simulink model "ProgettoIT"  (R2026b)
settings: Solver=VariableStepAuto  StopTime=3657
values from neighbouring files (symbols this model uses):
  m = sum(v .* dt) / Tstop    [excel.m]
  n = zeros(7,1)    [excel.m]
settings Model: Creator=francescocavazzoli  LastModifiedBy=Lorenzo

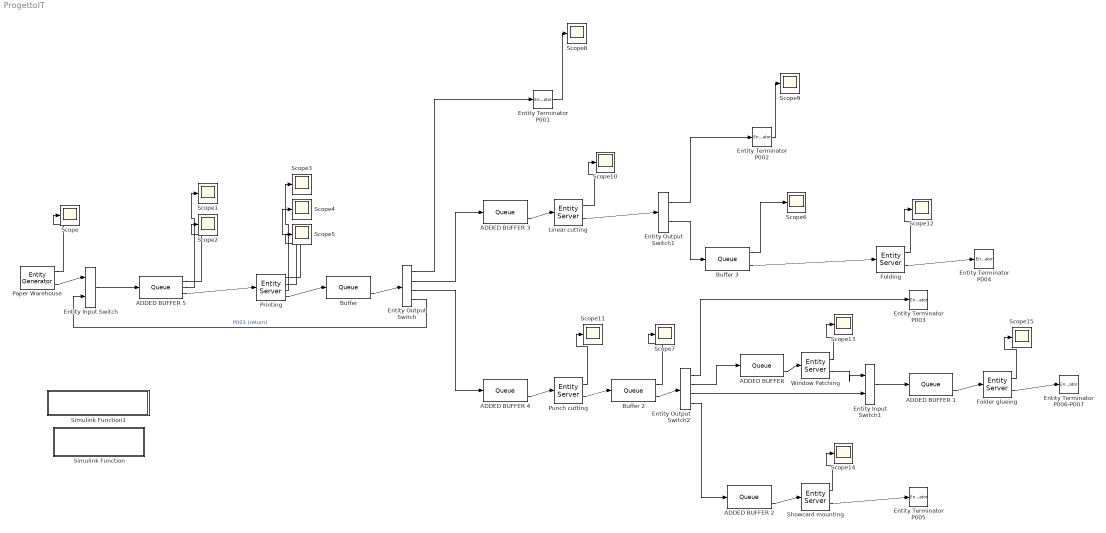
== system ProgettoIT ==
  ADDED BUFFER : Queue  InputPortMessageModes=m  OutputPortMessageModes=n,m  Capacity=inf  NumberEntitiesInBlock=on
      settings: OutputPortMap=o1,o5
  ADDED BUFFER {1..4} (4 alike) : Queue  InputPortMessageModes=m  OutputPortMessageModes=n,m  Capacity=inf  NumberEntitiesInBlock=on
      settings: OutputPortMap=o1,o5
  ADDED BUFFER 5 : Queue  InputPortMessageModes=m  OutputPortMessageModes=n,n,m  Capacity=inf  NumberEntitiesDeparted=on  NumberEntitiesInBlock=on
      settings: OutputPortMap=o0,o1,o5
  Buffer : Queue  InputPortMessageModes=m  OutputPortMessageModes=n,m  Capacity=inf  SortingDirection=Descending  NumberEntitiesInBlock=on
      settings: OutputPortMap=o1,o5
  Buffer 2 : Queue  InputPortMessageModes=m  OutputPortMessageModes=n,m  Capacity=inf  NumberEntitiesInBlock=on
      settings: OutputPortMap=o1,o5
  Buffer 3 : Queue  InputPortMessageModes=m  OutputPortMessageModes=n,m  Capacity=inf  NumberEntitiesInBlock=on
      settings: OutputPortMap=o1,o5
  Entity Input Switch : EntityInputSwitch  InputPortMessageModes=m,m  OutputPortMessageModes=m
  Entity Input Switch1 : EntityInputSwitch  InputPortMessageModes=m,m  OutputPortMessageModes=m
  Entity Output Switch : EntityOutputSwitch  InputPortMessageModes=m  OutputPortMessageModes=m,m,m,m  NumberOutputPorts=4  SwitchingCriterion=From attribute  SwitchAttributeName=OutPrint
      settings: OutputPortMap=o0,o1,o2,o3
  Entity Output Switch1 : EntityOutputSwitch  InputPortMessageModes=m  OutputPortMessageModes=m,m  SwitchingCriterion=From attribute  SwitchAttributeName=OutLin
  Entity Output Switch2 : EntityOutputSwitch  InputPortMessageModes=m  OutputPortMessageModes=m,m,m,m  NumberOutputPorts=4  SwitchingCriterion=From attribute  SwitchAttributeName=OutPunch
      settings: OutputPortMap=o0,o1,o2,o3
  Entity Terminator P001 : EntityTerminator  InputPortMessageModes=m  EntryAction=|  NumberEntitiesArrived=on
      | entity.FlowTime = ReadTime() - entity.Arrival;      % tempo di attraversamento [h]
      | Late = max(0, ReadTime() - entity.DueDate);          % ritardo rispetto al tempo max [h]
      | ToWorkspace(entity.Type, entity.FlowTime, Late);
      settings: OutputPortMap=o0
  Entity Terminator P002 : EntityTerminator  InputPortMessageModes=m  EntryAction=|  NumberEntitiesArrived=on
      | entity.FlowTime = ReadTime() - entity.Arrival;      % tempo di attraversamento [h]
      | Late = max(0, ReadTime() - entity.DueDate);          % ritardo rispetto al tempo max [h]
      | ToWorkspace(entity.Type, entity.FlowTime, Late);
      settings: OutputPortMap=o0
  "Entity Terminator P003 " : EntityTerminator  InputPortMessageModes=m  EntryAction=|
      | entity.FlowTime = ReadTime() - entity.Arrival;      % tempo di attraversamento [h]
      | Late = max(0, ReadTime() - entity.DueDate);          % ritardo rispetto al tempo max [h]
      | ToWorkspace(entity.Type, entity.FlowTime, Late);
  Entity Terminator P004 : EntityTerminator  InputPortMessageModes=m  EntryAction=|
      | entity.FlowTime = ReadTime() - entity.Arrival;      % tempo di attraversamento [h]
      | Late = max(0, ReadTime() - entity.DueDate);          % ritardo rispetto al tempo max [h]
      | ToWorkspace(entity.Type, entity.FlowTime, Late);
  "Entity Terminator P005 " : EntityTerminator  InputPortMessageModes=m  EntryAction=|
      | entity.FlowTime = ReadTime() - entity.Arrival;      % tempo di attraversamento [h]
      | Late = max(0, ReadTime() - entity.DueDate);          % ritardo rispetto al tempo max [h]
      | ToWorkspace(entity.Type, entity.FlowTime, Late);
  "Entity Terminator P006-P007 " : EntityTerminator  InputPortMessageModes=m  EntryAction=|
      | entity.FlowTime = ReadTime() - entity.Arrival;      % tempo di attraversamento [h]
      | Late = max(0, ReadTime() - entity.DueDate);          % ritardo rispetto al tempo max [h]
      | ToWorkspace(entity.Type, entity.FlowTime, Late);
  Folder glueing : EntityServer  InputPortMessageModes=m  OutputPortMessageModes=n,m  Capacity=2  ServiceTimeSource=MATLAB action  ServiceTimeAction=dt = (4 + entity.Pieces/54000)/0.5293;  Utilization=on
      settings: OutputPortMap=o5,o9
  Folding : EntityServer  InputPortMessageModes=m  OutputPortMessageModes=n,m  Capacity=3  ServiceTimeSource=MATLAB action  ServiceTimeAction=dt = (4 + entity.Pieces/5000)/0.5293;  Utilization=on
      settings: OutputPortMap=o5,o9
  Linear cutting : EntityServer  InputPortMessageModes=m  OutputPortMessageModes=n,m  Capacity=1  ServiceTimeSource=MATLAB action  ServiceTimeAction=dt = (0.5 + entity.Pieces/180000)/0.5293;  Utilization=on
      settings: OutputPortMap=o5,o9
  Paper Warehouse : EntityGenerator  OutputPortMessageModes=n,m  TimeSource=MATLAB action  IntergenerationTimeAction=|  GenerateAction=|  AttributeName=Pieces|Sheets|Type|Arrival|Pass|DueDate|OutPrint|OutLin|OutPunch|FlowTime  AttributeInitialValue=0|0|0|0|0|0|0|0|0|0  NumberEntitiesDeparted=on  EntityType=Structured  EntityTypeName=Entity
      IntergenerationTimeAction=|
      | coder.extrinsic('exprnd');
      | dt = 0.0; % Pre-allocazione per il compilatore
      | dt = exprnd(3657/600);
      GenerateAction=|
      | coder.extrinsic('randsample');
      | P = [0.15 0.03 0.42 0.04 0.05 0.23 0.08];        % % ordini P001..P007
      | S = [53333 53333 26667 50000 40000 24348 120000]; % fogli per ordine
      | T = [90 90 90 435 165 135 360];                   % tempo max di attraversamento [h]
      | type_val = 0; % Pre-allocazione per il compilatore
      | type_val = randsample(1:7, 1, true, P);
      | entity.Type = type_val;
      | entity.Sheets  = S(entity.Type);
      | entity.Pieces  = 18*entity.Sheets;
      | entity.Pass    = 0;
      | entity.Arrival = ReadTime();
      | entity.DueDate = entity.Arrival + T(entity.Type);
      | LP = [0 1 0 2 0 0 0];  entity.OutLin   = LP(entity.Type);  % dopo il taglio lineare: 1 = fine, 2 = piega
      | PU = [0 0 1 0 4 3 2];  entity.OutPunch = PU(entity.Type);  % dopo la fustella: 1 = fine, 2 = Finestratura, 3 = piega-incolla, 4 = owo
      settings: OutputPortMap=o0,o3
  Printing : EntityServer  InputPortMessageModes=m  OutputPortMessageModes=n,n,n,m  Capacity=3  ServiceTimeSource=MATLAB action  ServiceTimeValue=1/8000  ServiceTimeAction=dt = (5*20/60 + entity.Sheets/8000)/0.5293;  ServiceCompleteAction=|  NumberEntitiesDeparted=on  NumberEntitiesInBlock=on  Utilization=on
      | entity.Pass = entity.Pass + 1;
      | if entity.Type == 1 && entity.Pass == 1
      |     entity.OutPrint = 4;      % P001: ritorno in stampa
      | elseif entity.Type == 1
      |     entity.OutPrint = 1;      % P001 finito
      | elseif entity.Type == 2 || entity.Type == 4
      |     entity.OutPrint = 2;      % taglio lineare
      | else
      |     entity.OutPrint = 3;      % fustella
      | end
      settings: OutputPortMap=o0,o1,o5,o9
  "Punch cutting " : EntityServer  InputPortMessageModes=m  OutputPortMessageModes=n,m  Capacity=3  ServiceTimeSource=MATLAB action  ServiceTimeAction=dt = (2 + entity.Sheets/4000)/0.5293;  Utilization=on
      settings: OutputPortMap=o5,o9
  Scope{,1..15} (16 alike) : Scope
      Scope settings: ActiveDisplayYMinimum=-0.99999999999999956  ActiveDisplayYMaximum=19
      Scope10 settings: ActiveDisplayYMinimum=-0.024471490848986532  ActiveDisplayYMaximum=0.44643519443886448  DataLoggingVariableName=ScopeData10
      Scope11 settings: DataLoggingVariableName=ScopeData11
      Scope12 settings: ActiveDisplayYMinimum=0.25497380327143887  ActiveDisplayYMaximum=0.75796557224527028  DataLoggingVariableName=ScopeData12
      Scope13 settings: ActiveDisplayYMinimum=0.40962558539871696  ActiveDisplayYMaximum=0.68711566304961347  DataLoggingVariableName=ScopeData13
      Scope14 settings: ActiveDisplayYMinimum=0.075905038165493571  ActiveDisplayYMaximum=0.25791292970081553  DataLoggingVariableName=ScopeData14
      Scope15 settings: DataLoggingVariableName=ScopeData15
      Scope2 settings: DataLoggingVariableName=ScopeData2
      Scope3 settings: ActiveDisplayYMinimum=0.2405445003600471  ActiveDisplayYMaximum=1.0583804541198938  DataLoggingVariableName=ScopeData3
      Scope4 settings: DataLoggingVariableName=ScopeData4
      Scope5 settings: DataLoggingVariableName=ScopeData5
      Scope6 settings: DataLoggingVariableName=ScopeData6
      Scope7 settings: DataLoggingVariableName=ScopeData7
      Scope8 settings: DataLoggingVariableName=ScopeData8
      Scope9 settings: DataLoggingVariableName=ScopeData9
  Showcard mounting : EntityServer  InputPortMessageModes=m  OutputPortMessageModes=n,m  Capacity=1  ServiceTimeSource=MATLAB action  ServiceTimeAction=dt = (4 + entity.Pieces/54000)/0.5293;  Utilization=on
      settings: OutputPortMap=o5,o9
  Simulink Function : Subsystem  TreatAsAtomicUnit=on
  Simulink Function1 : Subsystem  TreatAsAtomicUnit=on
  Window Patching : EntityServer  InputPortMessageModes=m  OutputPortMessageModes=n,m  Capacity=2  ServiceTimeSource=MATLAB action  ServiceTimeAction=dt = (4 + entity.Pieces/54000)/0.5293;  Utilization=on
      settings: OutputPortMap=o5,o9
  wires:
  Printing/4 -> Buffer/1
  Buffer/2 -> Entity Output Switch/1
  Entity Output Switch/1 -> Entity Terminator P001/1
  Entity Output Switch/2 -> ADDED BUFFER 3/1
  Entity Output Switch/3 -> ADDED BUFFER 4/1
  Entity Output Switch/4 -> Entity Input Switch/2  "P001 (return)"
  Buffer 3/2 -> Folding/1
  Linear cutting/2 -> Entity Output Switch1/1
  Entity Output Switch1/2 -> Buffer 3/1
  Entity Output Switch1/1 -> Entity Terminator P002/1
  Entity Output Switch2/1 -> "Entity Terminator P003 "/1
  "Punch cutting "/2 -> Buffer 2/1
  Paper Warehouse/2 -> Entity Input Switch/1
  Buffer 2/2 -> Entity Output Switch2/1
  Entity Output Switch2/2 -> ADDED BUFFER/1
  Folding/2 -> Entity Terminator P004/1
  Window Patching/2 -> Entity Input Switch1/1
  Entity Input Switch1/1 -> ADDED BUFFER 1/1
  Entity Output Switch2/3 -> Entity Input Switch1/2
  Entity Output Switch2/4 -> ADDED BUFFER 2/1
  Folder glueing/2 -> "Entity Terminator P006-P007 "/1
  Showcard mounting/2 -> "Entity Terminator P005 "/1
  Paper Warehouse/1 -> Scope/1
  Printing/3 -> Scope3/1
  Printing/2 -> Scope4/1
  Printing/1 -> Scope5/1
  ADDED BUFFER 5/2 -> Scope1/1
  ADDED BUFFER 5/1 -> Scope2/1
  Entity Input Switch/1 -> ADDED BUFFER 5/1
  ADDED BUFFER 5/3 -> Printing/1
  Buffer 3/1 -> Scope6/1
  Buffer 2/1 -> Scope7/1
  Entity Terminator P001/1 -> Scope8/1
  Entity Terminator P002/1 -> Scope9/1
  ADDED BUFFER 3/2 -> Linear cutting/1
  ADDED BUFFER 4/2 -> "Punch cutting "/1
  Linear cutting/1 -> Scope10/1
  "Punch cutting "/1 -> Scope11/1
  Folding/1 -> Scope12/1
  Window Patching/1 -> Scope13/1
  Showcard mounting/1 -> Scope14/1
  Folder glueing/1 -> Scope15/1
  ADDED BUFFER/2 -> Window Patching/1
  ADDED BUFFER 2/2 -> Showcard mounting/1
  ADDED BUFFER 1/2 -> Folder glueing/1

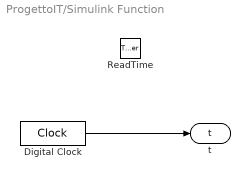
== system ProgettoIT/Simulink Function ==
  ReadTime : TriggerPort  TriggerType=function-call  IsSimulinkFunction=on  FunctionName=ReadTime  FunctionVisibility=scoped  VariantControl=(inherit)
  Digital Clock : DigitalClock  SampleTime=-1
  t : ArgOut  DisableCoverage=on  ArgumentName=t
  wires:
  Digital Clock/1 -> t/1

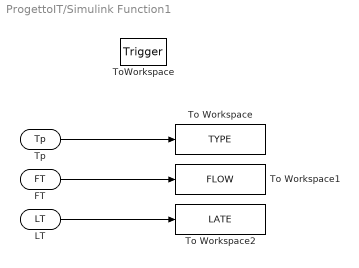
== system ProgettoIT/Simulink Function1 ==
  ToWorkspace : TriggerPort  TriggerType=function-call  IsSimulinkFunction=on  FunctionName=ToWorkspace  FunctionVisibility=scoped  VariantControl=(inherit)
  To Workspace : ToWorkspace  VariableName=TYPE  SaveFormat=Timeseries  SampleTime=-1
  To Workspace1 : ToWorkspace  VariableName=FLOW  SaveFormat=Timeseries  SampleTime=-1
  To Workspace2 : ToWorkspace  VariableName=LATE  SaveFormat=Timeseries  SampleTime=-1
  Tp : ArgIn  DisableCoverage=on  ArgumentName=Tp
  FT : ArgIn  Port=2  ArgumentName=FT
  LT : ArgIn  Port=3  ArgumentName=LT
  wires:
  Tp/1 -> To Workspace/1
  FT/1 -> To Workspace1/1
  LT/1 -> To Workspace2/1
